simulink model "MMC_phase_hackathon_circuit4_HAAS_20260216"  (R2024b)
settings: Solver=FixedStepDiscrete  StartTime=t_init_sim  StopTime=sim_time  FixedStep=Ts  RelTol=1e-3
values from neighbouring files (symbols this model uses):
  a = 1    [param_phase_circuit4_20260216.m]
  C1low1_active = 1    [script_MMC_phase_circuit4_twist_20260216.m]
  C2low1_active = 1    [script_MMC_phase_circuit4_twist_20260216.m]
  C_bus = 4400e-6    (= 0.0044)    [param_phase_circuit4_20260216.m]
  C_M_extra = C_m-twist_high_side_C    [param_phase_circuit4_20260216.m]
  duty_cycle = 0.95    [script_MMC_phase_circuit4_twist_20260216.m]
  f0 = 50    [param_phase_circuit4_20260216.m]
  feeder_current_lower_rate_limit = -10    [script_MMC_phase_circuit4_twist_20260216.m]    (also in twist_parameters.m = -500)
  feeder_current_tab = [0.328 0.217 0.162 0.132 0.109 0.094 0.083 0.075 0.068 0.062 0.058 0.054 ... (42 elements, 14x3)]    [feeder_current.mat]
  feeder_current_upper_rate_limit = 0.386/(20e-3)    (= 19.3)    [twist_parameters.m]
  is6VExternallySupplied = true    [script_MMC_phase_circuit4_twist_20260216.m]
  isFeederJumperOpen = true    [script_MMC_phase_circuit4_twist_20260216.m]
  L_arm = 60e-3    (= 0.06)    [param_phase_circuit4_20260216.m]
  m = 1    [param_phase_circuit4_20260216.m]
  N = 5    [param_phase_circuit4_20260216.m]
  power_losses = false    [script_MMC_phase_circuit4_twist_20260216.m]
  R = 15    [param_phase_circuit4_20260216.m]
  source_V = 0    [script_MMC_phase_circuit4_twist_20260216.m]
  time_charge = 0.1    [script_MMC_phase_circuit4_twist_20260216.m]
  time_decharge = 1.5    [script_MMC_phase_circuit4_twist_20260216.m]
  Ts = 5e-7    (= 5e-07)    [script_MMC_phase_circuit4_twist_20260216.m]
  twist_data_acquisition_delay = 50e-9    (= 5e-08)    [script_MMC_phase_circuit4_twist_20260216.m]    (also in twist_parameters.m)
  twist_data_sampling_period = 1/twist_freq_data_sampling    (= 5e-05)    [script_MMC_phase_circuit4_twist_20260216.m]    (also in twist_parameters.m)
  twist_dead_time = 200e-9    (= 2e-07)    [twist_parameters.m]
  twist_freq_switching = 200e3    (= 200000)    [twist_parameters.m]
  twist_high_side_adc_R = 1/(1/2e6 + 1/2e6 + 1/(330e3+5.6e3))    (= 251272.836178)    [twist_parameters.m]
  twist_high_side_C = 33e-6*4 + 4.7e-6*12    (= 0.0001884)    [twist_parameters.m]
  twist_high_side_feeder_R = 47e3+4.7e3    (= 51700)    [twist_parameters.m]
  twist_high_side_rC = 0.1    [twist_parameters.m]
  twist_low_side_adc_R = 150e3+470    (= 150470)    [twist_parameters.m]
  twist_low_side_C_ceramic = 3*4.7e-6    (= 1.41e-05)    [twist_parameters.m]
  twist_low_side_C_electrolytic = 47e-6    (= 4.7e-05)    [twist_parameters.m]
  twist_low_side_L = 33e-6    (= 3.3e-05)    [twist_parameters.m]
  twist_low_side_rC = 700e-3    (= 0.7)    [twist_parameters.m]
  twist_low_side_rL = 20e-3    (= 0.02)    [twist_parameters.m]
  twist_R_VCC = (tau_VCC/twist_high_side_C  - twist_high_side_rC)/(1-(tau_VCC/twist_high_side_C - twist_high_side_rC)/R_parallel)    (= 1110.74997822)    [twist_parameters.m]
  VDC = 48    [param_phase_circuit4_20260216.m]
undefined symbols (not defined in the file or in its folder): C_SM, feeder_current, gcbh, sps_rtmsupport, twist_low_side_lC
libraries: spsSeriesRLCBranchLib x135, spsTriangleGeneratorLib x60, spsMosfetLib x60, spsVoltageMeasurementLib x55, spsCurrentMeasurementLib x43, spsControlledCurrentSourceLib x30, spsDiodeLib x22, spsIdealSwitchLib x20, spsControlledVoltageSourceLib x1, spsGroundLib x1, spsMeanLib x1, spspowerguiLib x1
(part 17 of 18)

== system MMC_phase_hackathon_circuit4_HAAS_20260216/ /HB Twist M6/Twist Power Block/HRTimA_1/PWM Generator (2-Level)/Sampling/Sync Symmetrical/Sync_SymmetricalSampling/Sample & Hold ==
  In : Inport
  Enable : EnablePort
  Out : Outport  VectorParamsAs1DForOutWhenUnconnected=off
  wires:
  In/1 -> Out/1

== system MMC_phase_hackathon_circuit4_HAAS_20260216/ /HB Twist M6/Twist Power Block/HRTimA_2/PWM Generator (2-Level)/Sampling/Sync Symmetrical/Sync_SymmetricalSampling/Sample & Hold ==
  In : Inport
  Enable : EnablePort
  Out : Outport  VectorParamsAs1DForOutWhenUnconnected=off
  wires:
  In/1 -> Out/1

== system MMC_phase_hackathon_circuit4_HAAS_20260216/ /HB Twist M7/Twist Power Block/HRTimA_1/PWM Generator (2-Level)/Sampling/Sync Symmetrical/Sync_SymmetricalSampling/Sample & Hold ==
  In : Inport
  Enable : EnablePort
  Out : Outport  VectorParamsAs1DForOutWhenUnconnected=off
  wires:
  In/1 -> Out/1

== system MMC_phase_hackathon_circuit4_HAAS_20260216/ /HB Twist M7/Twist Power Block/HRTimA_2/PWM Generator (2-Level)/Sampling/Sync Symmetrical/Sync_SymmetricalSampling/Sample & Hold ==
  In : Inport
  Enable : EnablePort
  Out : Outport  VectorParamsAs1DForOutWhenUnconnected=off
  wires:
  In/1 -> Out/1

== system MMC_phase_hackathon_circuit4_HAAS_20260216/ /HB Twist M8/Twist Power Block/HRTimA_1/PWM Generator (2-Level)/Sampling/Sync Symmetrical/Sync_SymmetricalSampling/Sample & Hold ==
  In : Inport
  Enable : EnablePort
  Out : Outport  VectorParamsAs1DForOutWhenUnconnected=off
  wires:
  In/1 -> Out/1

== system MMC_phase_hackathon_circuit4_HAAS_20260216/ /HB Twist M8/Twist Power Block/HRTimA_2/PWM Generator (2-Level)/Sampling/Sync Symmetrical/Sync_SymmetricalSampling/Sample & Hold ==
  In : Inport
  Enable : EnablePort
  Out : Outport  VectorParamsAs1DForOutWhenUnconnected=off
  wires:
  In/1 -> Out/1

== system MMC_phase_hackathon_circuit4_HAAS_20260216/ /HB Twist M9/Twist Power Block/HRTimA_1/PWM Generator (2-Level)/Sampling/Sync Symmetrical/Sync_SymmetricalSampling/Sample & Hold ==
  In : Inport
  Enable : EnablePort
  Out : Outport  VectorParamsAs1DForOutWhenUnconnected=off
  wires:
  In/1 -> Out/1

== system MMC_phase_hackathon_circuit4_HAAS_20260216/ /HB Twist M9/Twist Power Block/HRTimA_2/PWM Generator (2-Level)/Sampling/Sync Symmetrical/Sync_SymmetricalSampling/Sample & Hold ==
  In : Inport
  Enable : EnablePort
  Out : Outport  VectorParamsAs1DForOutWhenUnconnected=off
  wires:
  In/1 -> Out/1

== matlab function MMC_phase_hackathon_circuit4_HAAS_20260216/ /HB Twist M3/Twist Power Block/Power losses branch 1/Branch DT loss ==
  data: twist_FET_Pdt output; ILow input
function twist_FET_Pdt = powerLossesDeadTime(ILow)
    %Twist gate power losses
    twist_freq_switching = 200e3;
    twist_FET_Vf = 1.2;
    twist_FET_tDr = 10e-9;
    twist_FET_tDf = 0;

    twist_FET_Pdt = twist_FET_Vf*ILow*(twist_FET_tDr+twist_FET_tDf)*twist_freq_switching;
end

== matlab function MMC_phase_hackathon_circuit4_HAAS_20260216/ /Sinus Modulation + Sorting Algorithm/Subsystem1/Tri phase/Tri2 ==
  data: ordre output; Vcp input; i input; sens output
function [ordre,sens] = fcn(Vcp, i)

[~, ordre] = sort(Vcp);

if i >= 0 
    sens = 1;
else 
    sens = 0;
end

% ordre = [1,2,3,4,5]';
% sens = 1;

== matlab function MMC_phase_hackathon_circuit4_HAAS_20260216/ /HB Twist M1/Twist Power Block/MATLAB Function ==
  data: i_feeder input; vC input; isfeederdisabled input; active_1 input; y output; Q_VCC output
function [y,Q_VCC]  = feeder_characteristics(i_feeder,vC,isfeederdisabled,active_1)

if(isfeederdisabled == 1)
    if(vC>=9.7)
        y = 11.2e-3;
        Q_VCC = 0;
    elseif(vC>=8.9 && vC < 9.7)
        if(active_1 == true)
            y = 11.2e-3;
            Q_VCC = 0;
        else
            y = 0;
            Q_VCC = 1;
        end
    else
        y = 0;
        Q_VCC = 1;
    end
else
    if(vC>=9.7)
        y = i_feeder;
        Q_VCC = 0;
    elseif(vC>=8.9 && vC < 9.7)
        if(active_1 == true)
            y = i_feeder;
            Q_VCC = 0;
        else
            y = 0;
            Q_VCC = 1;
        end
    else
        y = 0;
        Q_VCC = 1;
    end
end

== matlab function MMC_phase_hackathon_circuit4_HAAS_20260216/ /Sinus Modulation + Sorting Algorithm/Subsystem1/MATLAB Function2 ==
  data: ordre input; y output; sens input; N_on input; duty_cycle input
function y = fcn(ordre,sens,N_on,duty_cycle)

N_m = length(ordre);
Gp = zeros(1,N_m);
Ap0=ordre;

%% Sens positif (sens = 1)
if sens==1         % ON les condensateurs les moins chargés
    
    %K1 = 1 ; K2 = 0
    kp = 1:N_on;
    Gp(Ap0(kp))=duty_cycle;
    
    %K1 = 0 ; K2 = 1
    kp = N_on+1:N_m;
    Gp(Ap0(kp))=-0.01;

else            % ON les condensateurs les plus chargés
    
    %K1 = 1 ; K2 = 0
    kp = N_m:-1:N_m+1-N_on;
    Gp(Ap0(kp))=duty_cycle;

    %K1 = 0 ; K2 = 1
    kp = N_m-N_on:-1:1;
    Gp(Ap0(kp))=-0.01;

end
y=Gp;

== matlab function MMC_phase_hackathon_circuit4_HAAS_20260216/ /HB Twist M1/Twist Power Block/Power losses branch 1/Branch DT loss ==
  data: twist_FET_Pdt output; ILow input
function twist_FET_Pdt = powerLossesDeadTime(ILow)
    %Twist gate power losses
    twist_freq_switching = 200e3;
    twist_FET_Vf = 1.2;
    twist_FET_tDr = 10e-9;
    twist_FET_tDf = 0;

    twist_FET_Pdt = twist_FET_Vf*ILow*(twist_FET_tDr+twist_FET_tDf)*twist_freq_switching;
end

== matlab function MMC_phase_hackathon_circuit4_HAAS_20260216/ /HB Twist M1/Twist Power Block/Power losses branch 1/Branch cond loss ==
  data: twist_FET_Pcond output; VHigh input; VLow input; ILow input
function twist_FET_Pcond = powerLossesCond(VHigh, VLow, ILow)
    %Twist conduction power losses
    twist_FET_Ron = 0.025;

    twist_FET_PcondH = pow2(ILow)*twist_FET_Ron*(VLow/VHigh);
    twist_FET_PcondL = pow2(ILow)*twist_FET_Ron*(1 - VLow/VHigh);

    twist_FET_Pcond = twist_FET_PcondH + twist_FET_PcondL;
end

== matlab function MMC_phase_hackathon_circuit4_HAAS_20260216/ /HB Twist M1/Twist Power Block/Power losses branch 1/Branch gate loss ==
  data: twist_FET_Pg output
function twist_FET_Pg = powerLossesGate()
    %Twist gate power losses
    twist_freq_switching = 200e3;
    twist_FET_QgH = 31e-9;
    twist_FET_QgL = 31e-9;
    twist_FET_Vgs = 11;

    twist_FET_Pg = (twist_FET_QgH + twist_FET_QgL)*twist_FET_Vgs*twist_freq_switching;
end

== matlab function MMC_phase_hackathon_circuit4_HAAS_20260216/ /HB Twist M1/Twist Power Block/Power losses branch 1/Branch switching loss ==
  data: VHigh input; twist_FET_Psw output; ILow input
function twist_FET_Psw = powerLossesSwitch(VHigh, ILow)
    %Twist switch power losses
    twist_freq_switching = 200e3;
    twist_FET_trise = 17e-9;
    twist_FET_tfall = 9e-9;

    twist_FET_Psw = 1/2*VHigh*ILow*twist_freq_switching*(twist_FET_trise + twist_FET_tfall);
end

== matlab function MMC_phase_hackathon_circuit4_HAAS_20260216/ /HB Twist M1/Twist Power Block/Power losses branch 2/Branch DT loss ==
  data: twist_FET_Pdt output; ILow input
function twist_FET_Pdt = powerLossesDeadTime(ILow)
    %Twist gate power losses
    twist_freq_switching = 200e3;
    twist_FET_Vf = 1.2;
    twist_FET_tDr = 10e-9;
    twist_FET_tDf = 0;

    twist_FET_Pdt = twist_FET_Vf*ILow*(twist_FET_tDr+twist_FET_tDf)*twist_freq_switching;
end

== matlab function MMC_phase_hackathon_circuit4_HAAS_20260216/ /HB Twist M1/Twist Power Block/Power losses branch 2/Branch cond loss ==
  data: twist_FET_Pcond output; VHigh input; VLow input; ILow input
function twist_FET_Pcond = powerLossesCond(VHigh, VLow, ILow)
    %Twist conduction power losses
    twist_FET_Ron = 0.025;

    twist_FET_PcondH = pow2(ILow)*twist_FET_Ron*(VLow/VHigh);
    twist_FET_PcondL = pow2(ILow)*twist_FET_Ron*(1 - VLow/VHigh);

    twist_FET_Pcond = twist_FET_PcondH + twist_FET_PcondL;
end

== matlab function MMC_phase_hackathon_circuit4_HAAS_20260216/ /HB Twist M1/Twist Power Block/Power losses branch 2/Branch gate loss ==
  data: twist_FET_Pg output
function twist_FET_Pg = powerLossesGate()
    %Twist gate power losses
    twist_freq_switching = 200e3;
    twist_FET_QgH = 31e-9;
    twist_FET_QgL = 31e-9;
    twist_FET_Vgs = 11;

    twist_FET_Pg = (twist_FET_QgH + twist_FET_QgL)*twist_FET_Vgs*twist_freq_switching;
end

== matlab function MMC_phase_hackathon_circuit4_HAAS_20260216/ /HB Twist M2/Twist Power Block/MATLAB Function ==
  data: i_feeder input; vC input; isfeederdisabled input; active_1 input; y output; Q_VCC output
function [y,Q_VCC]  = feeder_characteristics(i_feeder,vC,isfeederdisabled,active_1)

if(isfeederdisabled == 1)
    if(vC>=9.7)
        y = 11.2e-3;
        Q_VCC = 0;
    elseif(vC>=8.9 && vC < 9.7)
        if(active_1 == true)
            y = 11.2e-3;
            Q_VCC = 0;
        else
            y = 0;
            Q_VCC = 1;
        end
    else
        y = 0;
        Q_VCC = 1;
    end
else
    if(vC>=9.7)
        y = i_feeder;
        Q_VCC = 0;
    elseif(vC>=8.9 && vC < 9.7)
        if(active_1 == true)
            y = i_feeder;
            Q_VCC = 0;
        else
            y = 0;
            Q_VCC = 1;
        end
    else
        y = 0;
        Q_VCC = 1;
    end
end

== matlab function MMC_phase_hackathon_circuit4_HAAS_20260216/ /HB Twist M1/Twist Power Block/Power losses branch 2/Branch switching loss ==
  data: VHigh input; twist_FET_Psw output; ILow input
function twist_FET_Psw = powerLossesSwitch(VHigh, ILow)
    %Twist switch power losses
    twist_freq_switching = 200e3;
    twist_FET_trise = 17e-9;
    twist_FET_tfall = 9e-9;

    twist_FET_Psw = 1/2*VHigh*ILow*twist_freq_switching*(twist_FET_trise + twist_FET_tfall);
end

== matlab function MMC_phase_hackathon_circuit4_HAAS_20260216/ /HB Twist M3/Twist Power Block/Power losses branch 1/Branch cond loss ==
  data: twist_FET_Pcond output; VHigh input; VLow input; ILow input
function twist_FET_Pcond = powerLossesCond(VHigh, VLow, ILow)
    %Twist conduction power losses
    twist_FET_Ron = 0.025;

    twist_FET_PcondH = pow2(ILow)*twist_FET_Ron*(VLow/VHigh);
    twist_FET_PcondL = pow2(ILow)*twist_FET_Ron*(1 - VLow/VHigh);

    twist_FET_Pcond = twist_FET_PcondH + twist_FET_PcondL;
end

== matlab function MMC_phase_hackathon_circuit4_HAAS_20260216/ /HB Twist M3/Twist Power Block/Power losses branch 1/Branch gate loss ==
  data: twist_FET_Pg output
function twist_FET_Pg = powerLossesGate()
    %Twist gate power losses
    twist_freq_switching = 200e3;
    twist_FET_QgH = 31e-9;
    twist_FET_QgL = 31e-9;
    twist_FET_Vgs = 11;

    twist_FET_Pg = (twist_FET_QgH + twist_FET_QgL)*twist_FET_Vgs*twist_freq_switching;
end

== matlab function MMC_phase_hackathon_circuit4_HAAS_20260216/ /HB Twist M3/Twist Power Block/Power losses branch 1/Branch switching loss ==
  data: VHigh input; twist_FET_Psw output; ILow input
function twist_FET_Psw = powerLossesSwitch(VHigh, ILow)
    %Twist switch power losses
    twist_freq_switching = 200e3;
    twist_FET_trise = 17e-9;
    twist_FET_tfall = 9e-9;

    twist_FET_Psw = 1/2*VHigh*ILow*twist_freq_switching*(twist_FET_trise + twist_FET_tfall);
end

== matlab function MMC_phase_hackathon_circuit4_HAAS_20260216/ /HB Twist M3/Twist Power Block/Power losses branch 2/Branch DT loss ==
  data: twist_FET_Pdt output; ILow input
function twist_FET_Pdt = powerLossesDeadTime(ILow)
    %Twist gate power losses
    twist_freq_switching = 200e3;
    twist_FET_Vf = 1.2;
    twist_FET_tDr = 10e-9;
    twist_FET_tDf = 0;

    twist_FET_Pdt = twist_FET_Vf*ILow*(twist_FET_tDr+twist_FET_tDf)*twist_freq_switching;
end

== matlab function MMC_phase_hackathon_circuit4_HAAS_20260216/ /HB Twist M3/Twist Power Block/Power losses branch 2/Branch cond loss ==
  data: twist_FET_Pcond output; VHigh input; VLow input; ILow input
function twist_FET_Pcond = powerLossesCond(VHigh, VLow, ILow)
    %Twist conduction power losses
    twist_FET_Ron = 0.025;

    twist_FET_PcondH = pow2(ILow)*twist_FET_Ron*(VLow/VHigh);
    twist_FET_PcondL = pow2(ILow)*twist_FET_Ron*(1 - VLow/VHigh);

    twist_FET_Pcond = twist_FET_PcondH + twist_FET_PcondL;
end

== matlab function MMC_phase_hackathon_circuit4_HAAS_20260216/ /HB Twist M3/Twist Power Block/Power losses branch 2/Branch gate loss ==
  data: twist_FET_Pg output
function twist_FET_Pg = powerLossesGate()
    %Twist gate power losses
    twist_freq_switching = 200e3;
    twist_FET_QgH = 31e-9;
    twist_FET_QgL = 31e-9;
    twist_FET_Vgs = 11;

    twist_FET_Pg = (twist_FET_QgH + twist_FET_QgL)*twist_FET_Vgs*twist_freq_switching;
end

== matlab function MMC_phase_hackathon_circuit4_HAAS_20260216/ /HB Twist M3/Twist Power Block/Power losses branch 2/Branch switching loss ==
  data: VHigh input; twist_FET_Psw output; ILow input
function twist_FET_Psw = powerLossesSwitch(VHigh, ILow)
    %Twist switch power losses
    twist_freq_switching = 200e3;
    twist_FET_trise = 17e-9;
    twist_FET_tfall = 9e-9;

    twist_FET_Psw = 1/2*VHigh*ILow*twist_freq_switching*(twist_FET_trise + twist_FET_tfall);
end

== matlab function MMC_phase_hackathon_circuit4_HAAS_20260216/ /HB Twist M4/Twist Power Block/MATLAB Function ==
  data: i_feeder input; vC input; isfeederdisabled input; active_1 input; y output; Q_VCC output
function [y,Q_VCC]  = feeder_characteristics(i_feeder,vC,isfeederdisabled,active_1)

if(isfeederdisabled == 1)
    if(vC>=9.7)
        y = 11.2e-3;
        Q_VCC = 0;
    elseif(vC>=8.9 && vC < 9.7)
        if(active_1 == true)
            y = 11.2e-3;
            Q_VCC = 0;
        else
            y = 0;
            Q_VCC = 1;
        end
    else
        y = 0;
        Q_VCC = 1;
    end
else
    if(vC>=9.7)
        y = i_feeder;
        Q_VCC = 0;
    elseif(vC>=8.9 && vC < 9.7)
        if(active_1 == true)
            y = i_feeder;
            Q_VCC = 0;
        else
            y = 0;
            Q_VCC = 1;
        end
    else
        y = 0;
        Q_VCC = 1;
    end
end

== matlab function MMC_phase_hackathon_circuit4_HAAS_20260216/ /HB Twist M4/Twist Power Block/Power losses branch 1/Branch DT loss ==
  data: twist_FET_Pdt output; ILow input
function twist_FET_Pdt = powerLossesDeadTime(ILow)
    %Twist gate power losses
    twist_freq_switching = 200e3;
    twist_FET_Vf = 1.2;
    twist_FET_tDr = 10e-9;
    twist_FET_tDf = 0;

    twist_FET_Pdt = twist_FET_Vf*ILow*(twist_FET_tDr+twist_FET_tDf)*twist_freq_switching;
end

== matlab function MMC_phase_hackathon_circuit4_HAAS_20260216/ /HB Twist M4/Twist Power Block/Power losses branch 1/Branch cond loss ==
  data: twist_FET_Pcond output; VHigh input; VLow input; ILow input
function twist_FET_Pcond = powerLossesCond(VHigh, VLow, ILow)
    %Twist conduction power losses
    twist_FET_Ron = 0.025;

    twist_FET_PcondH = pow2(ILow)*twist_FET_Ron*(VLow/VHigh);
    twist_FET_PcondL = pow2(ILow)*twist_FET_Ron*(1 - VLow/VHigh);

    twist_FET_Pcond = twist_FET_PcondH + twist_FET_PcondL;
end

== matlab function MMC_phase_hackathon_circuit4_HAAS_20260216/ /HB Twist M4/Twist Power Block/Power losses branch 1/Branch gate loss ==
  data: twist_FET_Pg output
function twist_FET_Pg = powerLossesGate()
    %Twist gate power losses
    twist_freq_switching = 200e3;
    twist_FET_QgH = 31e-9;
    twist_FET_QgL = 31e-9;
    twist_FET_Vgs = 11;

    twist_FET_Pg = (twist_FET_QgH + twist_FET_QgL)*twist_FET_Vgs*twist_freq_switching;
end

== matlab function MMC_phase_hackathon_circuit4_HAAS_20260216/ /HB Twist M4/Twist Power Block/Power losses branch 1/Branch switching loss ==
  data: VHigh input; twist_FET_Psw output; ILow input
function twist_FET_Psw = powerLossesSwitch(VHigh, ILow)
    %Twist switch power losses
    twist_freq_switching = 200e3;
    twist_FET_trise = 17e-9;
    twist_FET_tfall = 9e-9;

    twist_FET_Psw = 1/2*VHigh*ILow*twist_freq_switching*(twist_FET_trise + twist_FET_tfall);
end

== matlab function MMC_phase_hackathon_circuit4_HAAS_20260216/ /HB Twist M4/Twist Power Block/Power losses branch 2/Branch DT loss ==
  data: twist_FET_Pdt output; ILow input
function twist_FET_Pdt = powerLossesDeadTime(ILow)
    %Twist gate power losses
    twist_freq_switching = 200e3;
    twist_FET_Vf = 1.2;
    twist_FET_tDr = 10e-9;
    twist_FET_tDf = 0;

    twist_FET_Pdt = twist_FET_Vf*ILow*(twist_FET_tDr+twist_FET_tDf)*twist_freq_switching;
end

== matlab function MMC_phase_hackathon_circuit4_HAAS_20260216/ /HB Twist M4/Twist Power Block/Power losses branch 2/Branch cond loss ==
  data: twist_FET_Pcond output; VHigh input; VLow input; ILow input
function twist_FET_Pcond = powerLossesCond(VHigh, VLow, ILow)
    %Twist conduction power losses
    twist_FET_Ron = 0.025;

    twist_FET_PcondH = pow2(ILow)*twist_FET_Ron*(VLow/VHigh);
    twist_FET_PcondL = pow2(ILow)*twist_FET_Ron*(1 - VLow/VHigh);

    twist_FET_Pcond = twist_FET_PcondH + twist_FET_PcondL;
end

== matlab function MMC_phase_hackathon_circuit4_HAAS_20260216/ /HB Twist M2/Twist Power Block/Power losses branch 1/Branch DT loss ==
  data: twist_FET_Pdt output; ILow input
function twist_FET_Pdt = powerLossesDeadTime(ILow)
    %Twist gate power losses
    twist_freq_switching = 200e3;
    twist_FET_Vf = 1.2;
    twist_FET_tDr = 10e-9;
    twist_FET_tDf = 0;

    twist_FET_Pdt = twist_FET_Vf*ILow*(twist_FET_tDr+twist_FET_tDf)*twist_freq_switching;
end

== matlab function MMC_phase_hackathon_circuit4_HAAS_20260216/ /HB Twist M4/Twist Power Block/Power losses branch 2/Branch gate loss ==
  data: twist_FET_Pg output
function twist_FET_Pg = powerLossesGate()
    %Twist gate power losses
    twist_freq_switching = 200e3;
    twist_FET_QgH = 31e-9;
    twist_FET_QgL = 31e-9;
    twist_FET_Vgs = 11;

    twist_FET_Pg = (twist_FET_QgH + twist_FET_QgL)*twist_FET_Vgs*twist_freq_switching;
end

== matlab function MMC_phase_hackathon_circuit4_HAAS_20260216/ /HB Twist M4/Twist Power Block/Power losses branch 2/Branch switching loss ==
  data: VHigh input; twist_FET_Psw output; ILow input
function twist_FET_Psw = powerLossesSwitch(VHigh, ILow)
    %Twist switch power losses
    twist_freq_switching = 200e3;
    twist_FET_trise = 17e-9;
    twist_FET_tfall = 9e-9;

    twist_FET_Psw = 1/2*VHigh*ILow*twist_freq_switching*(twist_FET_trise + twist_FET_tfall);
end

== matlab function MMC_phase_hackathon_circuit4_HAAS_20260216/ /HB Twist M5/Twist Power Block/MATLAB Function ==
  data: i_feeder input; vC input; isfeederdisabled input; active_1 input; y output; Q_VCC output
function [y,Q_VCC]  = feeder_characteristics(i_feeder,vC,isfeederdisabled,active_1)

if(isfeederdisabled == 1)
    if(vC>=9.7)
        y = 11.2e-3;
        Q_VCC = 0;
    elseif(vC>=8.9 && vC < 9.7)
        if(active_1 == true)
            y = 11.2e-3;
            Q_VCC = 0;
        else
            y = 0;
            Q_VCC = 1;
        end
    else
        y = 0;
        Q_VCC = 1;
    end
else
    if(vC>=9.7)
        y = i_feeder;
        Q_VCC = 0;
    elseif(vC>=8.9 && vC < 9.7)
        if(active_1 == true)
            y = i_feeder;
            Q_VCC = 0;
        else
            y = 0;
            Q_VCC = 1;
        end
    else
        y = 0;
        Q_VCC = 1;
    end
end

== matlab function MMC_phase_hackathon_circuit4_HAAS_20260216/ /HB Twist M5/Twist Power Block/Power losses branch 1/Branch DT loss ==
  data: twist_FET_Pdt output; ILow input
function twist_FET_Pdt = powerLossesDeadTime(ILow)
    %Twist gate power losses
    twist_freq_switching = 200e3;
    twist_FET_Vf = 1.2;
    twist_FET_tDr = 10e-9;
    twist_FET_tDf = 0;

    twist_FET_Pdt = twist_FET_Vf*ILow*(twist_FET_tDr+twist_FET_tDf)*twist_freq_switching;
end

== matlab function MMC_phase_hackathon_circuit4_HAAS_20260216/ /HB Twist M5/Twist Power Block/Power losses branch 1/Branch cond loss ==
  data: twist_FET_Pcond output; VHigh input; VLow input; ILow input
function twist_FET_Pcond = powerLossesCond(VHigh, VLow, ILow)
    %Twist conduction power losses
    twist_FET_Ron = 0.025;

    twist_FET_PcondH = pow2(ILow)*twist_FET_Ron*(VLow/VHigh);
    twist_FET_PcondL = pow2(ILow)*twist_FET_Ron*(1 - VLow/VHigh);

    twist_FET_Pcond = twist_FET_PcondH + twist_FET_PcondL;
end

== matlab function MMC_phase_hackathon_circuit4_HAAS_20260216/ /HB Twist M5/Twist Power Block/Power losses branch 1/Branch gate loss ==
  data: twist_FET_Pg output
function twist_FET_Pg = powerLossesGate()
    %Twist gate power losses
    twist_freq_switching = 200e3;
    twist_FET_QgH = 31e-9;
    twist_FET_QgL = 31e-9;
    twist_FET_Vgs = 11;

    twist_FET_Pg = (twist_FET_QgH + twist_FET_QgL)*twist_FET_Vgs*twist_freq_switching;
end

== matlab function MMC_phase_hackathon_circuit4_HAAS_20260216/ /HB Twist M5/Twist Power Block/Power losses branch 1/Branch switching loss ==
  data: VHigh input; twist_FET_Psw output; ILow input
function twist_FET_Psw = powerLossesSwitch(VHigh, ILow)
    %Twist switch power losses
    twist_freq_switching = 200e3;
    twist_FET_trise = 17e-9;
    twist_FET_tfall = 9e-9;

    twist_FET_Psw = 1/2*VHigh*ILow*twist_freq_switching*(twist_FET_trise + twist_FET_tfall);
end

== matlab function MMC_phase_hackathon_circuit4_HAAS_20260216/ /HB Twist M5/Twist Power Block/Power losses branch 2/Branch DT loss ==
  data: twist_FET_Pdt output; ILow input
function twist_FET_Pdt = powerLossesDeadTime(ILow)
    %Twist gate power losses
    twist_freq_switching = 200e3;
    twist_FET_Vf = 1.2;
    twist_FET_tDr = 10e-9;
    twist_FET_tDf = 0;

    twist_FET_Pdt = twist_FET_Vf*ILow*(twist_FET_tDr+twist_FET_tDf)*twist_freq_switching;
end

== matlab function MMC_phase_hackathon_circuit4_HAAS_20260216/ /HB Twist M2/Twist Power Block/Power losses branch 1/Branch cond loss ==
  data: twist_FET_Pcond output; VHigh input; VLow input; ILow input
function twist_FET_Pcond = powerLossesCond(VHigh, VLow, ILow)
    %Twist conduction power losses
    twist_FET_Ron = 0.025;

    twist_FET_PcondH = pow2(ILow)*twist_FET_Ron*(VLow/VHigh);
    twist_FET_PcondL = pow2(ILow)*twist_FET_Ron*(1 - VLow/VHigh);

    twist_FET_Pcond = twist_FET_PcondH + twist_FET_PcondL;
end

== matlab function MMC_phase_hackathon_circuit4_HAAS_20260216/ /HB Twist M5/Twist Power Block/Power losses branch 2/Branch cond loss ==
  data: twist_FET_Pcond output; VHigh input; VLow input; ILow input
function twist_FET_Pcond = powerLossesCond(VHigh, VLow, ILow)
    %Twist conduction power losses
    twist_FET_Ron = 0.025;

    twist_FET_PcondH = pow2(ILow)*twist_FET_Ron*(VLow/VHigh);
    twist_FET_PcondL = pow2(ILow)*twist_FET_Ron*(1 - VLow/VHigh);

    twist_FET_Pcond = twist_FET_PcondH + twist_FET_PcondL;
end

== matlab function MMC_phase_hackathon_circuit4_HAAS_20260216/ /HB Twist M5/Twist Power Block/Power losses branch 2/Branch gate loss ==
  data: twist_FET_Pg output
function twist_FET_Pg = powerLossesGate()
    %Twist gate power losses
    twist_freq_switching = 200e3;
    twist_FET_QgH = 31e-9;
    twist_FET_QgL = 31e-9;
    twist_FET_Vgs = 11;

    twist_FET_Pg = (twist_FET_QgH + twist_FET_QgL)*twist_FET_Vgs*twist_freq_switching;
end

== matlab function MMC_phase_hackathon_circuit4_HAAS_20260216/ /HB Twist M5/Twist Power Block/Power losses branch 2/Branch switching loss ==
  data: VHigh input; twist_FET_Psw output; ILow input
function twist_FET_Psw = powerLossesSwitch(VHigh, ILow)
    %Twist switch power losses
    twist_freq_switching = 200e3;
    twist_FET_trise = 17e-9;
    twist_FET_tfall = 9e-9;

    twist_FET_Psw = 1/2*VHigh*ILow*twist_freq_switching*(twist_FET_trise + twist_FET_tfall);
end

== matlab function MMC_phase_hackathon_circuit4_HAAS_20260216/ /Sinus Modulation + Sorting Algorithm/Subsystem2/MATLAB Function2 ==
  data: ordre input; y output; sens input; N_on input; duty_cycle input
function y = fcn(ordre,sens,N_on,duty_cycle)

N_m = length(ordre);
Gp = zeros(1,N_m);
Ap0=ordre;

%% Sens positif (sens = 1)
if sens==1         % ON les condensateurs les moins chargés
    
    %K1 = 1 ; K2 = 0
    kp = 1:N_on;
    Gp(Ap0(kp))=duty_cycle;
    
    %K1 = 0 ; K2 = 1
    kp = N_on+1:N_m;
    Gp(Ap0(kp))=-0.01;

else            % ON les condensateurs les plus chargés
    
    %K1 = 1 ; K2 = 0
    kp = N_m:-1:N_m+1-N_on;
    Gp(Ap0(kp))=duty_cycle;

    %K1 = 0 ; K2 = 1
    kp = N_m-N_on:-1:1;
    Gp(Ap0(kp))=-0.01;

end
y=Gp;

== matlab function MMC_phase_hackathon_circuit4_HAAS_20260216/ /Sinus Modulation + Sorting Algorithm/Subsystem2/Tri phase/Tri2 ==
  data: ordre output; Vcp input; i input; sens output
function [ordre,sens] = fcn(Vcp, i)

[~, ordre] = sort(Vcp);

if i >= 0 
    sens = 1;
else 
    sens = 0;
end

% ordre = [1,2,3,4,5]';
% sens = 1;

== matlab function MMC_phase_hackathon_circuit4_HAAS_20260216/ /HB Twist M10/Twist Power Block/MATLAB Function ==
  data: i_feeder input; vC input; isfeederdisabled input; active_1 input; y output; Q_VCC output
function [y,Q_VCC]  = feeder_characteristics(i_feeder,vC,isfeederdisabled,active_1)

if(isfeederdisabled == 1)
    if(vC>=9.7)
        y = 11.2e-3;
        Q_VCC = 0;
    elseif(vC>=8.9 && vC < 9.7)
        if(active_1 == true)
            y = 11.2e-3;
            Q_VCC = 0;
        else
            y = 0;
            Q_VCC = 1;
        end
    else
        y = 0;
        Q_VCC = 1;
    end
else
    if(vC>=9.7)
        y = i_feeder;
        Q_VCC = 0;
    elseif(vC>=8.9 && vC < 9.7)
        if(active_1 == true)
            y = i_feeder;
            Q_VCC = 0;
        else
            y = 0;
            Q_VCC = 1;
        end
    else
        y = 0;
        Q_VCC = 1;
    end
end

== matlab function MMC_phase_hackathon_circuit4_HAAS_20260216/ /HB Twist M10/Twist Power Block/Power losses branch 1/Branch DT loss ==
  data: twist_FET_Pdt output; ILow input
function twist_FET_Pdt = powerLossesDeadTime(ILow)
    %Twist gate power losses
    twist_freq_switching = 200e3;
    twist_FET_Vf = 1.2;
    twist_FET_tDr = 10e-9;
    twist_FET_tDf = 0;

    twist_FET_Pdt = twist_FET_Vf*ILow*(twist_FET_tDr+twist_FET_tDf)*twist_freq_switching;
end

== matlab function MMC_phase_hackathon_circuit4_HAAS_20260216/ /HB Twist M10/Twist Power Block/Power losses branch 1/Branch cond loss ==
  data: twist_FET_Pcond output; VHigh input; VLow input; ILow input
function twist_FET_Pcond = powerLossesCond(VHigh, VLow, ILow)
    %Twist conduction power losses
    twist_FET_Ron = 0.025;

    twist_FET_PcondH = pow2(ILow)*twist_FET_Ron*(VLow/VHigh);
    twist_FET_PcondL = pow2(ILow)*twist_FET_Ron*(1 - VLow/VHigh);

    twist_FET_Pcond = twist_FET_PcondH + twist_FET_PcondL;
end

== matlab function MMC_phase_hackathon_circuit4_HAAS_20260216/ /HB Twist M10/Twist Power Block/Power losses branch 1/Branch gate loss ==
  data: twist_FET_Pg output
function twist_FET_Pg = powerLossesGate()
    %Twist gate power losses
    twist_freq_switching = 200e3;
    twist_FET_QgH = 31e-9;
    twist_FET_QgL = 31e-9;
    twist_FET_Vgs = 11;

    twist_FET_Pg = (twist_FET_QgH + twist_FET_QgL)*twist_FET_Vgs*twist_freq_switching;
end

== matlab function MMC_phase_hackathon_circuit4_HAAS_20260216/ /HB Twist M10/Twist Power Block/Power losses branch 1/Branch switching loss ==
  data: VHigh input; twist_FET_Psw output; ILow input
function twist_FET_Psw = powerLossesSwitch(VHigh, ILow)
    %Twist switch power losses
    twist_freq_switching = 200e3;
    twist_FET_trise = 17e-9;
    twist_FET_tfall = 9e-9;

    twist_FET_Psw = 1/2*VHigh*ILow*twist_freq_switching*(twist_FET_trise + twist_FET_tfall);
end

== matlab function MMC_phase_hackathon_circuit4_HAAS_20260216/ /HB Twist M10/Twist Power Block/Power losses branch 2/Branch DT loss ==
  data: twist_FET_Pdt output; ILow input
function twist_FET_Pdt = powerLossesDeadTime(ILow)
    %Twist gate power losses
    twist_freq_switching = 200e3;
    twist_FET_Vf = 1.2;
    twist_FET_tDr = 10e-9;
    twist_FET_tDf = 0;

    twist_FET_Pdt = twist_FET_Vf*ILow*(twist_FET_tDr+twist_FET_tDf)*twist_freq_switching;
end

== matlab function MMC_phase_hackathon_circuit4_HAAS_20260216/ /HB Twist M2/Twist Power Block/Power losses branch 1/Branch gate loss ==
  data: twist_FET_Pg output
function twist_FET_Pg = powerLossesGate()
    %Twist gate power losses
    twist_freq_switching = 200e3;
    twist_FET_QgH = 31e-9;
    twist_FET_QgL = 31e-9;
    twist_FET_Vgs = 11;

    twist_FET_Pg = (twist_FET_QgH + twist_FET_QgL)*twist_FET_Vgs*twist_freq_switching;
end

== matlab function MMC_phase_hackathon_circuit4_HAAS_20260216/ /HB Twist M10/Twist Power Block/Power losses branch 2/Branch cond loss ==
  data: twist_FET_Pcond output; VHigh input; VLow input; ILow input
function twist_FET_Pcond = powerLossesCond(VHigh, VLow, ILow)
    %Twist conduction power losses
    twist_FET_Ron = 0.025;

    twist_FET_PcondH = pow2(ILow)*twist_FET_Ron*(VLow/VHigh);
    twist_FET_PcondL = pow2(ILow)*twist_FET_Ron*(1 - VLow/VHigh);

    twist_FET_Pcond = twist_FET_PcondH + twist_FET_PcondL;
end

== matlab function MMC_phase_hackathon_circuit4_HAAS_20260216/ /HB Twist M10/Twist Power Block/Power losses branch 2/Branch gate loss ==
  data: twist_FET_Pg output
function twist_FET_Pg = powerLossesGate()
    %Twist gate power losses
    twist_freq_switching = 200e3;
    twist_FET_QgH = 31e-9;
    twist_FET_QgL = 31e-9;
    twist_FET_Vgs = 11;

    twist_FET_Pg = (twist_FET_QgH + twist_FET_QgL)*twist_FET_Vgs*twist_freq_switching;
end

== matlab function MMC_phase_hackathon_circuit4_HAAS_20260216/ /HB Twist M10/Twist Power Block/Power losses branch 2/Branch switching loss ==
  data: VHigh input; twist_FET_Psw output; ILow input
function twist_FET_Psw = powerLossesSwitch(VHigh, ILow)
    %Twist switch power losses
    twist_freq_switching = 200e3;
    twist_FET_trise = 17e-9;
    twist_FET_tfall = 9e-9;

    twist_FET_Psw = 1/2*VHigh*ILow*twist_freq_switching*(twist_FET_trise + twist_FET_tfall);
end

== matlab function MMC_phase_hackathon_circuit4_HAAS_20260216/ /HB Twist M6/Twist Power Block/MATLAB Function ==
  data: i_feeder input; vC input; isfeederdisabled input; active_1 input; y output; Q_VCC output
function [y,Q_VCC]  = feeder_characteristics(i_feeder,vC,isfeederdisabled,active_1)

if(isfeederdisabled == 1)
    if(vC>=9.7)
        y = 11.2e-3;
        Q_VCC = 0;
    elseif(vC>=8.9 && vC < 9.7)
        if(active_1 == true)
            y = 11.2e-3;
            Q_VCC = 0;
        else
            y = 0;
            Q_VCC = 1;
        end
    else
        y = 0;
        Q_VCC = 1;
    end
else
    if(vC>=9.7)
        y = i_feeder;
        Q_VCC = 0;
    elseif(vC>=8.9 && vC < 9.7)
        if(active_1 == true)
            y = i_feeder;
            Q_VCC = 0;
        else
            y = 0;
            Q_VCC = 1;
        end
    else
        y = 0;
        Q_VCC = 1;
    end
end

== matlab function MMC_phase_hackathon_circuit4_HAAS_20260216/ /HB Twist M6/Twist Power Block/Power losses branch 1/Branch DT loss ==
  data: twist_FET_Pdt output; ILow input
function twist_FET_Pdt = powerLossesDeadTime(ILow)
    %Twist gate power losses
    twist_freq_switching = 200e3;
    twist_FET_Vf = 1.2;
    twist_FET_tDr = 10e-9;
    twist_FET_tDf = 0;

    twist_FET_Pdt = twist_FET_Vf*ILow*(twist_FET_tDr+twist_FET_tDf)*twist_freq_switching;
end

== matlab function MMC_phase_hackathon_circuit4_HAAS_20260216/ /HB Twist M6/Twist Power Block/Power losses branch 1/Branch cond loss ==
  data: twist_FET_Pcond output; VHigh input; VLow input; ILow input
function twist_FET_Pcond = powerLossesCond(VHigh, VLow, ILow)
    %Twist conduction power losses
    twist_FET_Ron = 0.025;

    twist_FET_PcondH = pow2(ILow)*twist_FET_Ron*(VLow/VHigh);
    twist_FET_PcondL = pow2(ILow)*twist_FET_Ron*(1 - VLow/VHigh);

    twist_FET_Pcond = twist_FET_PcondH + twist_FET_PcondL;
end

== matlab function MMC_phase_hackathon_circuit4_HAAS_20260216/ /HB Twist M6/Twist Power Block/Power losses branch 1/Branch gate loss ==
  data: twist_FET_Pg output
function twist_FET_Pg = powerLossesGate()
    %Twist gate power losses
    twist_freq_switching = 200e3;
    twist_FET_QgH = 31e-9;
    twist_FET_QgL = 31e-9;
    twist_FET_Vgs = 11;

    twist_FET_Pg = (twist_FET_QgH + twist_FET_QgL)*twist_FET_Vgs*twist_freq_switching;
end

== matlab function MMC_phase_hackathon_circuit4_HAAS_20260216/ /HB Twist M6/Twist Power Block/Power losses branch 1/Branch switching loss ==
  data: VHigh input; twist_FET_Psw output; ILow input
function twist_FET_Psw = powerLossesSwitch(VHigh, ILow)
    %Twist switch power losses
    twist_freq_switching = 200e3;
    twist_FET_trise = 17e-9;
    twist_FET_tfall = 9e-9;

    twist_FET_Psw = 1/2*VHigh*ILow*twist_freq_switching*(twist_FET_trise + twist_FET_tfall);
end

== matlab function MMC_phase_hackathon_circuit4_HAAS_20260216/ /HB Twist M2/Twist Power Block/Power losses branch 1/Branch switching loss ==
  data: VHigh input; twist_FET_Psw output; ILow input
function twist_FET_Psw = powerLossesSwitch(VHigh, ILow)
    %Twist switch power losses
    twist_freq_switching = 200e3;
    twist_FET_trise = 17e-9;
    twist_FET_tfall = 9e-9;

    twist_FET_Psw = 1/2*VHigh*ILow*twist_freq_switching*(twist_FET_trise + twist_FET_tfall);
end

== matlab function MMC_phase_hackathon_circuit4_HAAS_20260216/ /HB Twist M6/Twist Power Block/Power losses branch 2/Branch DT loss ==
  data: twist_FET_Pdt output; ILow input
function twist_FET_Pdt = powerLossesDeadTime(ILow)
    %Twist gate power losses
    twist_freq_switching = 200e3;
    twist_FET_Vf = 1.2;
    twist_FET_tDr = 10e-9;
    twist_FET_tDf = 0;

    twist_FET_Pdt = twist_FET_Vf*ILow*(twist_FET_tDr+twist_FET_tDf)*twist_freq_switching;
end

== matlab function MMC_phase_hackathon_circuit4_HAAS_20260216/ /HB Twist M6/Twist Power Block/Power losses branch 2/Branch cond loss ==
  data: twist_FET_Pcond output; VHigh input; VLow input; ILow input
function twist_FET_Pcond = powerLossesCond(VHigh, VLow, ILow)
    %Twist conduction power losses
    twist_FET_Ron = 0.025;

    twist_FET_PcondH = pow2(ILow)*twist_FET_Ron*(VLow/VHigh);
    twist_FET_PcondL = pow2(ILow)*twist_FET_Ron*(1 - VLow/VHigh);

    twist_FET_Pcond = twist_FET_PcondH + twist_FET_PcondL;
end

== matlab function MMC_phase_hackathon_circuit4_HAAS_20260216/ /HB Twist M6/Twist Power Block/Power losses branch 2/Branch gate loss ==
  data: twist_FET_Pg output
function twist_FET_Pg = powerLossesGate()
    %Twist gate power losses
    twist_freq_switching = 200e3;
    twist_FET_QgH = 31e-9;
    twist_FET_QgL = 31e-9;
    twist_FET_Vgs = 11;

    twist_FET_Pg = (twist_FET_QgH + twist_FET_QgL)*twist_FET_Vgs*twist_freq_switching;
end

== matlab function MMC_phase_hackathon_circuit4_HAAS_20260216/ /HB Twist M6/Twist Power Block/Power losses branch 2/Branch switching loss ==
  data: VHigh input; twist_FET_Psw output; ILow input
function twist_FET_Psw = powerLossesSwitch(VHigh, ILow)
    %Twist switch power losses
    twist_freq_switching = 200e3;
    twist_FET_trise = 17e-9;
    twist_FET_tfall = 9e-9;

    twist_FET_Psw = 1/2*VHigh*ILow*twist_freq_switching*(twist_FET_trise + twist_FET_tfall);
end

== matlab function MMC_phase_hackathon_circuit4_HAAS_20260216/ /HB Twist M7/Twist Power Block/MATLAB Function ==
  data: i_feeder input; vC input; isfeederdisabled input; active_1 input; y output; Q_VCC output
function [y,Q_VCC]  = feeder_characteristics(i_feeder,vC,isfeederdisabled,active_1)

if(isfeederdisabled == 1)
    if(vC>=9.7)
        y = 11.2e-3;
        Q_VCC = 0;
    elseif(vC>=8.9 && vC < 9.7)
        if(active_1 == true)
            y = 11.2e-3;
            Q_VCC = 0;
        else
            y = 0;
            Q_VCC = 1;
        end
    else
        y = 0;
        Q_VCC = 1;
    end
else
    if(vC>=9.7)
        y = i_feeder;
        Q_VCC = 0;
    elseif(vC>=8.9 && vC < 9.7)
        if(active_1 == true)
            y = i_feeder;
            Q_VCC = 0;
        else
            y = 0;
            Q_VCC = 1;
        end
    else
        y = 0;
        Q_VCC = 1;
    end
end

== matlab function MMC_phase_hackathon_circuit4_HAAS_20260216/ /HB Twist M7/Twist Power Block/Power losses branch 1/Branch DT loss ==
  data: twist_FET_Pdt output; ILow input
function twist_FET_Pdt = powerLossesDeadTime(ILow)
    %Twist gate power losses
    twist_freq_switching = 200e3;
    twist_FET_Vf = 1.2;
    twist_FET_tDr = 10e-9;
    twist_FET_tDf = 0;

    twist_FET_Pdt = twist_FET_Vf*ILow*(twist_FET_tDr+twist_FET_tDf)*twist_freq_switching;
end

== matlab function MMC_phase_hackathon_circuit4_HAAS_20260216/ /HB Twist M7/Twist Power Block/Power losses branch 1/Branch cond loss ==
  data: twist_FET_Pcond output; VHigh input; VLow input; ILow input
function twist_FET_Pcond = powerLossesCond(VHigh, VLow, ILow)
    %Twist conduction power losses
    twist_FET_Ron = 0.025;

    twist_FET_PcondH = pow2(ILow)*twist_FET_Ron*(VLow/VHigh);
    twist_FET_PcondL = pow2(ILow)*twist_FET_Ron*(1 - VLow/VHigh);

    twist_FET_Pcond = twist_FET_PcondH + twist_FET_PcondL;
end

== matlab function MMC_phase_hackathon_circuit4_HAAS_20260216/ /HB Twist M7/Twist Power Block/Power losses branch 1/Branch gate loss ==
  data: twist_FET_Pg output
function twist_FET_Pg = powerLossesGate()
    %Twist gate power losses
    twist_freq_switching = 200e3;
    twist_FET_QgH = 31e-9;
    twist_FET_QgL = 31e-9;
    twist_FET_Vgs = 11;

    twist_FET_Pg = (twist_FET_QgH + twist_FET_QgL)*twist_FET_Vgs*twist_freq_switching;
end

== matlab function MMC_phase_hackathon_circuit4_HAAS_20260216/ /HB Twist M7/Twist Power Block/Power losses branch 1/Branch switching loss ==
  data: VHigh input; twist_FET_Psw output; ILow input
function twist_FET_Psw = powerLossesSwitch(VHigh, ILow)
    %Twist switch power losses
    twist_freq_switching = 200e3;
    twist_FET_trise = 17e-9;
    twist_FET_tfall = 9e-9;

    twist_FET_Psw = 1/2*VHigh*ILow*twist_freq_switching*(twist_FET_trise + twist_FET_tfall);
end

== matlab function MMC_phase_hackathon_circuit4_HAAS_20260216/ /HB Twist M7/Twist Power Block/Power losses branch 2/Branch DT loss ==
  data: twist_FET_Pdt output; ILow input
function twist_FET_Pdt = powerLossesDeadTime(ILow)
    %Twist gate power losses
    twist_freq_switching = 200e3;
    twist_FET_Vf = 1.2;
    twist_FET_tDr = 10e-9;
    twist_FET_tDf = 0;

    twist_FET_Pdt = twist_FET_Vf*ILow*(twist_FET_tDr+twist_FET_tDf)*twist_freq_switching;
end

== matlab function MMC_phase_hackathon_circuit4_HAAS_20260216/ /HB Twist M2/Twist Power Block/Power losses branch 2/Branch DT loss ==
  data: twist_FET_Pdt output; ILow input
function twist_FET_Pdt = powerLossesDeadTime(ILow)
    %Twist gate power losses
    twist_freq_switching = 200e3;
    twist_FET_Vf = 1.2;
    twist_FET_tDr = 10e-9;
    twist_FET_tDf = 0;

    twist_FET_Pdt = twist_FET_Vf*ILow*(twist_FET_tDr+twist_FET_tDf)*twist_freq_switching;
end

== matlab function MMC_phase_hackathon_circuit4_HAAS_20260216/ /HB Twist M7/Twist Power Block/Power losses branch 2/Branch cond loss ==
  data: twist_FET_Pcond output; VHigh input; VLow input; ILow input
function twist_FET_Pcond = powerLossesCond(VHigh, VLow, ILow)
    %Twist conduction power losses
    twist_FET_Ron = 0.025;

    twist_FET_PcondH = pow2(ILow)*twist_FET_Ron*(VLow/VHigh);
    twist_FET_PcondL = pow2(ILow)*twist_FET_Ron*(1 - VLow/VHigh);

    twist_FET_Pcond = twist_FET_PcondH + twist_FET_PcondL;
end

== matlab function MMC_phase_hackathon_circuit4_HAAS_20260216/ /HB Twist M7/Twist Power Block/Power losses branch 2/Branch gate loss ==
  data: twist_FET_Pg output
function twist_FET_Pg = powerLossesGate()
    %Twist gate power losses
    twist_freq_switching = 200e3;
    twist_FET_QgH = 31e-9;
    twist_FET_QgL = 31e-9;
    twist_FET_Vgs = 11;

    twist_FET_Pg = (twist_FET_QgH + twist_FET_QgL)*twist_FET_Vgs*twist_freq_switching;
end

== matlab function MMC_phase_hackathon_circuit4_HAAS_20260216/ /HB Twist M7/Twist Power Block/Power losses branch 2/Branch switching loss ==
  data: VHigh input; twist_FET_Psw output; ILow input
function twist_FET_Psw = powerLossesSwitch(VHigh, ILow)
    %Twist switch power losses
    twist_freq_switching = 200e3;
    twist_FET_trise = 17e-9;
    twist_FET_tfall = 9e-9;

    twist_FET_Psw = 1/2*VHigh*ILow*twist_freq_switching*(twist_FET_trise + twist_FET_tfall);
end

== matlab function MMC_phase_hackathon_circuit4_HAAS_20260216/ /HB Twist M8/Twist Power Block/MATLAB Function ==
  data: i_feeder input; vC input; isfeederdisabled input; active_1 input; y output; Q_VCC output
function [y,Q_VCC]  = feeder_characteristics(i_feeder,vC,isfeederdisabled,active_1)

if(isfeederdisabled == 1)
    if(vC>=9.7)
        y = 11.2e-3;
        Q_VCC = 0;
    elseif(vC>=8.9 && vC < 9.7)
        if(active_1 == true)
            y = 11.2e-3;
            Q_VCC = 0;
        else
            y = 0;
            Q_VCC = 1;
        end
    else
        y = 0;
        Q_VCC = 1;
    end
else
    if(vC>=9.7)
        y = i_feeder;
        Q_VCC = 0;
    elseif(vC>=8.9 && vC < 9.7)
        if(active_1 == true)
            y = i_feeder;
            Q_VCC = 0;
        else
            y = 0;
            Q_VCC = 1;
        end
    else
        y = 0;
        Q_VCC = 1;
    end
end

== matlab function MMC_phase_hackathon_circuit4_HAAS_20260216/ /HB Twist M8/Twist Power Block/Power losses branch 1/Branch DT loss ==
  data: twist_FET_Pdt output; ILow input
function twist_FET_Pdt = powerLossesDeadTime(ILow)
    %Twist gate power losses
    twist_freq_switching = 200e3;
    twist_FET_Vf = 1.2;
    twist_FET_tDr = 10e-9;
    twist_FET_tDf = 0;

    twist_FET_Pdt = twist_FET_Vf*ILow*(twist_FET_tDr+twist_FET_tDf)*twist_freq_switching;
end

== matlab function MMC_phase_hackathon_circuit4_HAAS_20260216/ /HB Twist M8/Twist Power Block/Power losses branch 1/Branch cond loss ==
  data: twist_FET_Pcond output; VHigh input; VLow input; ILow input
function twist_FET_Pcond = powerLossesCond(VHigh, VLow, ILow)
    %Twist conduction power losses
    twist_FET_Ron = 0.025;

    twist_FET_PcondH = pow2(ILow)*twist_FET_Ron*(VLow/VHigh);
    twist_FET_PcondL = pow2(ILow)*twist_FET_Ron*(1 - VLow/VHigh);

    twist_FET_Pcond = twist_FET_PcondH + twist_FET_PcondL;
end

== matlab function MMC_phase_hackathon_circuit4_HAAS_20260216/ /HB Twist M8/Twist Power Block/Power losses branch 1/Branch gate loss ==
  data: twist_FET_Pg output
function twist_FET_Pg = powerLossesGate()
    %Twist gate power losses
    twist_freq_switching = 200e3;
    twist_FET_QgH = 31e-9;
    twist_FET_QgL = 31e-9;
    twist_FET_Vgs = 11;

    twist_FET_Pg = (twist_FET_QgH + twist_FET_QgL)*twist_FET_Vgs*twist_freq_switching;
end

== matlab function MMC_phase_hackathon_circuit4_HAAS_20260216/ /HB Twist M8/Twist Power Block/Power losses branch 1/Branch switching loss ==
  data: VHigh input; twist_FET_Psw output; ILow input
function twist_FET_Psw = powerLossesSwitch(VHigh, ILow)
    %Twist switch power losses
    twist_freq_switching = 200e3;
    twist_FET_trise = 17e-9;
    twist_FET_tfall = 9e-9;

    twist_FET_Psw = 1/2*VHigh*ILow*twist_freq_switching*(twist_FET_trise + twist_FET_tfall);
end

== matlab function MMC_phase_hackathon_circuit4_HAAS_20260216/ /HB Twist M8/Twist Power Block/Power losses branch 2/Branch DT loss ==
  data: twist_FET_Pdt output; ILow input
function twist_FET_Pdt = powerLossesDeadTime(ILow)
    %Twist gate power losses
    twist_freq_switching = 200e3;
    twist_FET_Vf = 1.2;
    twist_FET_tDr = 10e-9;
    twist_FET_tDf = 0;

    twist_FET_Pdt = twist_FET_Vf*ILow*(twist_FET_tDr+twist_FET_tDf)*twist_freq_switching;
end

== matlab function MMC_phase_hackathon_circuit4_HAAS_20260216/ /HB Twist M2/Twist Power Block/Power losses branch 2/Branch cond loss ==
  data: twist_FET_Pcond output; VHigh input; VLow input; ILow input
function twist_FET_Pcond = powerLossesCond(VHigh, VLow, ILow)
    %Twist conduction power losses
    twist_FET_Ron = 0.025;

    twist_FET_PcondH = pow2(ILow)*twist_FET_Ron*(VLow/VHigh);
    twist_FET_PcondL = pow2(ILow)*twist_FET_Ron*(1 - VLow/VHigh);

    twist_FET_Pcond = twist_FET_PcondH + twist_FET_PcondL;
end

== matlab function MMC_phase_hackathon_circuit4_HAAS_20260216/ /HB Twist M8/Twist Power Block/Power losses branch 2/Branch cond loss ==
  data: twist_FET_Pcond output; VHigh input; VLow input; ILow input
function twist_FET_Pcond = powerLossesCond(VHigh, VLow, ILow)
    %Twist conduction power losses
    twist_FET_Ron = 0.025;

    twist_FET_PcondH = pow2(ILow)*twist_FET_Ron*(VLow/VHigh);
    twist_FET_PcondL = pow2(ILow)*twist_FET_Ron*(1 - VLow/VHigh);

    twist_FET_Pcond = twist_FET_PcondH + twist_FET_PcondL;
end

== matlab function MMC_phase_hackathon_circuit4_HAAS_20260216/ /HB Twist M8/Twist Power Block/Power losses branch 2/Branch gate loss ==
  data: twist_FET_Pg output
function twist_FET_Pg = powerLossesGate()
    %Twist gate power losses
    twist_freq_switching = 200e3;
    twist_FET_QgH = 31e-9;
    twist_FET_QgL = 31e-9;
    twist_FET_Vgs = 11;

    twist_FET_Pg = (twist_FET_QgH + twist_FET_QgL)*twist_FET_Vgs*twist_freq_switching;
end

== matlab function MMC_phase_hackathon_circuit4_HAAS_20260216/ /HB Twist M8/Twist Power Block/Power losses branch 2/Branch switching loss ==
  data: VHigh input; twist_FET_Psw output; ILow input
function twist_FET_Psw = powerLossesSwitch(VHigh, ILow)
    %Twist switch power losses
    twist_freq_switching = 200e3;
    twist_FET_trise = 17e-9;
    twist_FET_tfall = 9e-9;

    twist_FET_Psw = 1/2*VHigh*ILow*twist_freq_switching*(twist_FET_trise + twist_FET_tfall);
end

== matlab function MMC_phase_hackathon_circuit4_HAAS_20260216/ /HB Twist M9/Twist Power Block/MATLAB Function ==
  data: i_feeder input; vC input; isfeederdisabled input; active_1 input; y output; Q_VCC output
function [y,Q_VCC]  = feeder_characteristics(i_feeder,vC,isfeederdisabled,active_1)

if(isfeederdisabled == 1)
    if(vC>=9.7)
        y = 11.2e-3;
        Q_VCC = 0;
    elseif(vC>=8.9 && vC < 9.7)
        if(active_1 == true)
            y = 11.2e-3;
            Q_VCC = 0;
        else
            y = 0;
            Q_VCC = 1;
        end
    else
        y = 0;
        Q_VCC = 1;
    end
else
    if(vC>=9.7)
        y = i_feeder;
        Q_VCC = 0;
    elseif(vC>=8.9 && vC < 9.7)
        if(active_1 == true)
            y = i_feeder;
            Q_VCC = 0;
        else
            y = 0;
            Q_VCC = 1;
        end
    else
        y = 0;
        Q_VCC = 1;
    end
end

== matlab function MMC_phase_hackathon_circuit4_HAAS_20260216/ /HB Twist M9/Twist Power Block/Power losses branch 1/Branch DT loss ==
  data: twist_FET_Pdt output; ILow input
function twist_FET_Pdt = powerLossesDeadTime(ILow)
    %Twist gate power losses
    twist_freq_switching = 200e3;
    twist_FET_Vf = 1.2;
    twist_FET_tDr = 10e-9;
    twist_FET_tDf = 0;

    twist_FET_Pdt = twist_FET_Vf*ILow*(twist_FET_tDr+twist_FET_tDf)*twist_freq_switching;
end
